simulink library "ASEToolBox2023a"  (R2023a)
settings: Solver=ode45  StartTime=0.0  StopTime=10.0  RelTol=1e-3  EnableMultiTasking=on
values from neighbouring files (symbols this model uses):
  dt = get_param(gcbh, 'g_output_datatype')    [maskSysComCallbacks_Receive.m]    (also in maskSysComCallbacks_Send.m = get_param(gcbh, 'g_input_datatype'))
undefined symbols (not defined in the file or in its folder): dCx, dCy, dCz, DiscIntNeverNeededParam, Discrete, dmassX, dmassY, dmassZ, dMx, dMy, dMz, dp, dp0, dp1, dp2, dp3, lmd_high, lmd_low, magnitude, Newton, p0, p1, p2, p3, p4, phi0, phi000, phi1, phi2, phi3, phi4, r1, r2, r3, r4, Raphson, theta0, theta1, theta2, theta3, theta4, Time, u0, u1, u2, u3, v0, v0_max, v0_min, v1, v111, v2, v222, v3, v333, v4, W1, w1, w2, W2 ... (+2)
libraries: simulink x38, etargetslib x28, simulink_extras x5, slpidlib x2, ctrlSharedLib x2, aerolibatmos2 x1, aerolibconvert2 x1, aerolibtransform2 x1, sharedtransform x1, dspstat3 x1, dspsolvers x1
(part 2 of 6)

== system ASEToolBox2023a/Aerocraft Model/ACE Guidance and Control Algorithm ==
  Time : Inport
  Eular : Inport  Port=2
  Wxyz1 : Inport  Port=3
  H : Inport  Port=4
  Add : Sum  Inputs=+-
  Add1 : Sum  Inputs=+-
  Add2 : Sum  Inputs=+-
  Add3 : Sum
  DeltaXC : Constant  Value=0
  DeltaYC : Constant  Value=0
  Discrete Transfer Fcn : DiscreteTransferFcn  Numerator=[0.0309]  Denominator=[1 -0.9691]
  Gain : Gain  Gain=0
  Gain1 : Gain
  Gain2 : Gain
  Lookup Table : Lookup  InitFcn=|  InputValues=phi000(:,1)  Table=phi000(:,2)  SaturateOnIntegerOverflow=off
      | phi00=[0.0 	60
      | 0.5 	53.175
      | 1.0 	47.6
      | 1.5 	43.275
      | 2.0 	40.2
      | 2.5 	39.1055
      | 3.0 	38.012
      | 3.5 	36.9195
      | 4.0 	35.828
      | 4.5 	34.7375
      | 5.0 	33.648
      | 5.5 	32.5595
      | 6.0 	31.472
      | 6.5 	30.3855
      | 7.0 	29.3
      | 7.5 	28.2155
      | 8.0 	27.132
      | 8.5 	26.0495
      | 9.0 	24.968
      | 9.5 	23.8875
      | 10.0 	22.808
      | 10.5 	21.7295
      | 11.0 	20.652
      | 11.5 	19.5755
      | 12.0 	18.5
      | 12.5 	17.4255
      | 13.0 	16.352
      | 13.5 	15.2795
      | 14.0 	14.208
      | 14.5 	13.1375
      | 15.0 	12.068
      | 15.5 	10.9995
      | 16.0 	9.932
      | 16.5 	8.8655
      | 17.0 	7.8
      | 17.5 	6.7355
      | 18.0 	5.672
      | 18.5 	4.6095
      | 19.0 	3.548
      | 19.5 	2.4875
      | 20.0 	1.428
      | 20.5 	0.3695
      | 21.0 	-0.688
      | 21.5 	-1.7445
      | 22.0 	-2.8
      | 22.5 	-3.8545
      | 23.0 	-4.908
      | 23.5 	-5.9605
      | 24.0 	-7.012
      | 24.5 	-8.0625
      | 25.0 	-9.112
      | 25.5 	-10.1605
      | 26.0 	-11.208
      | 26.5 	-12.2545
      | 27.0 	-13.3
      | 27.5 	-14.3445
      | 28.0 	-15.388
      | 28.5 	-14.862975
      | 29.0 	-14.3379
      | 29.5 	-13.812775
      | 30.0 	-13.2876
      | 30.5 	-12.762375
      | 31.0 	-12.2371
      | 31.5 	-11.711775
      | 32.0 	-11.1864
      | 32.5 	-10.660975
      | 33.0 	-10.1355
      | 33.5 	-9.609975
      | 34.0 	-9.0844
      | 34.5 	-8.558775
      | 35.0 	-8.0331
      | 35.5 	-7.507375
      | 36.0 	-6.9816
      | 36.5 	-6.455775
      | 37.0 	-5.9299
      | 37.5 	-5.403975
      | 38.0 	-4.878
      | 38.5 	-4.351975
      | 39.0 	-3.8259
      | 39.5 	-3.299775
      | 40.0 	-2.7736
      | 40.5 	-2.247375
      | 41.0 	-1.7211
      | 41.5 	-1.194775
      | 42.0 	-0.6684
      | 42.5 	-0.141975
      | 43.0 	0.3845
      | 43.5 	0.911025
      | 44.0 	1.4376
      | 44.5 	1.964225
      | 45.0 	2.4909
      | 45.5 	3.0167
      | 46.0 	3.01485
      | 46.5 	3.0133
      | 47.0 	3.01205
      | 47.5 	3.0111
      | 48.0 	3.01045
      | 48.5 	3.0101
      | 49.0 	3.01005
      | 49.5 	3.0103
      | 50.0 	3.01085
      | 50.5 	3.0117
      | 51.0 	3.01285
      | 51.5 	3.0143
      | 52.0 	3.01605
      | 52.5 	3.0181
      | 53.0 	3.02045
      | 53.5 	3.0231
      | 54.0 	3.02605
      | 54.5 	3.0293
      | 55.0 	3.03285
      | 55.5 	3.0367
      | 56.0 	3.04085
      | 56.5 	3.0453
      | 57.0 	3.05005
      | 57.5 	3.0551
      | 58.0 	3.06045
      | 58.5 	3.0661
      | 59.0 	3.07205
      | 59.5 	3.0783
      | 60.0 	3.08485
      | 60.5 	3.0917
      | 61.0 	3.09885
      | 61.5 	3.1063
      | 62.0 	3.11405
      | 62.5 	3.1221
      | 63.0 	3.13045
      | 63.5 	3.1391
      | 64.0 	3.14805
      | 64.5 	3.1573
      | 65.0 	3.16685
      | 65.5 	3.1767
      | 66.0 	3.18685
      | 66.5 	3.1973
      | 67.0 	3.20805
      | 67.5 	3.2191
      | 68.0 	3.23045
      | 68.5 	3.2421
      | 69.0 	3.25405
      | 69.5 	3.2663
      | 70.0 	3.27885
      | 70.5 	3.2917
      | 71.0 	3.30485
      | 71.5 	3.3183
      | 72.0 	3.33205
      | 72.5 	3.3461
      | 73.0 	3.36045
      | 73.5 	3.3751
      | 74.0 	3.39005
      | 74.5 	3.4053
      | 75.0 	3.42085
      | 75.5 	3.4367
      | 76.0 	3.45285
      | 76.5 	3.4693
      | 77.0 	3.48605
      | 77.5 	3.5031
      | 78.0 	3.52045
      | 78.5 	3.5381
      | 79.0 	3.55605
      | 79.5 	3.5743
      | 80.0 	3.59285
      | 80.5 	3.6117
      | 81.0 	3.63085
      | 81.5 	3.6503
      | 82.0 	3.67005
      | 82.5 	3.6901
      | 83.0 	3.71045
      | 83.5 	3.7311
      | 84.0 	3.75205
      | 84.5 	3.7733
      | 85.0 	3.79485
      | 85.5 	3.8167
      | 86.0 	3.83885
      | 86.5 	3.8613
      | 87.0 	3.88405
      | 87.5 	3.9071
      | 88.0 	3.93045
      | 88.5 	3.9541
      | 89.0 	3.97805
      | 89.5 	4.0023
      | 90.0 	4.02685
      | 90.5 	4.0517
      | 91.0 	4.07685
      | 91.5 	4.1023
      | 92.0 	4.12805
      | 92.5 	4.1541
      | 93.0 	4.18045
      | 93.5 	4.2071
      | 94.0 	4.23405
      | 94.5 	4.2613
      | 95.0 	4.28885
      | 95.5 	4.3167
      | 96.0 	4.34485
      | 96.5 	4.3733
      | 97.0 	4.40205
      | 97.5 	4.4311
      | 98.0 	4.46045
      | 98.5 	4.4901
      | 99.0 	4.52005
      | 99.5 	4.5503
      | 100.0 	4.5808
      | 100.5 	5.4608
      | 101.0 	6.3008
      | 101.5 	7.1008
      | 102.0 	7.8608
      | 102.5 	8.5808
      | 103.0 	9.2608
      | 103.5 	9.9008
      | 104.0 	10.5008
      | 104.5 	11.0608
      | 105.0 	11.5808
      | 105.5 	12.0608
      | 106.0 	12.5008
      | 106.5 	12.9008
      | 107.0 	13.2608
      | 107.5 	13.5808
      | 108.0 	13.8608
      | 108.5 	14.1008
      | 109.0 	14.3008
      | 109.5 	14.4608
      | 110.0 	14.5808
      | 110.5 	14.6608
      | 111.0 	14.7008
      | 111.5 	14.7008
      | 112.0 	14.6608
      | 112.5 	14.5808
      | 113.0 	14.4608
      | 113.5 	14.3008
      | 114.0 	14.1008
      | 114.5 	13.8608
      | 115.0 	13.5808
      | 115.5 	13.2608
      | 116.0 	12.9008
      | 116.5 	12.5008
      | 117.0 	12.0608
      | 117.5 	11.5808
      | 118.0 	11.0608
      | 118.5 	10.5008
      | 119.0 	9.9008
      | 119.5 	9.2608
      | 120.0 	8.5808
      | 120.5 	7.8608
      | 121.0 	7.1008
      | 121.5 	6.3008
      | 122.0 	5.4608
      | 122.5 	4.5808
      | 123.0 	3.6608
      | 123.5 	2.7008
      | 124.0 	1.7008
      | 124.5 	0.6608
      | 125.0 	-0.4192
      | 125.5 	-1.5392
      | 126.0 	-2.6992
      | 126.5 	-3.8992
      | 127.0 	-5.1392
      | 127.5 	-6.4192
      | 128.0 	-7.7392
      | 128.5 	-9.0992
      | 129.0 	-10.4992
      | 129.5 	-11.9392
      | 130.0 	-13.4192
      | 130.5 	-14.9392
      | 131.0 	-16.4992
      | 131.5 	-18.0992
      | 132.0 	-19.7392
      | 132.5 	-21.4192
      | 133.0 	-23.1392
      | 133.5 	-24.8992
      | 134.0 	-26.6992
      | 134.5 	-28.5392
      | 135.0 	-30.4192
      | 135.5 	-32.3392
      | 136.0 	-34.2992
      | 136.5 	-36.2992
      | 137.0 	-38.3392
      | 137.5 	-40.4192];
  Lookup Table1 : Lookup  InitFcn=|  InputValues=[0:1:137]  Table=|  SaturateOnIntegerOverflow=off
      InitFcn=|
      | phi00=[0.0 	60
      | 0.5 	53.175
      | 1.0 	47.6
      | 1.5 	43.275
      | 2.0 	40.2
      | 2.5 	39.1055
      | 3.0 	38.012
      | 3.5 	36.9195
      | 4.0 	35.828
      | 4.5 	34.7375
      | 5.0 	33.648
      | 5.5 	32.5595
      | 6.0 	31.472
      | 6.5 	30.3855
      | 7.0 	29.3
      | 7.5 	28.2155
      | 8.0 	27.132
      | 8.5 	26.0495
      | 9.0 	24.968
      | 9.5 	23.8875
      | 10.0 	22.808
      | 10.5 	21.7295
      | 11.0 	20.652
      | 11.5 	19.5755
      | 12.0 	18.5
      | 12.5 	17.4255
      | 13.0 	16.352
      | 13.5 	15.2795
      | 14.0 	14.208
      | 14.5 	13.1375
      | 15.0 	12.068
      | 15.5 	10.9995
      | 16.0 	9.932
      | 16.5 	8.8655
      | 17.0 	7.8
      | 17.5 	6.7355
      | 18.0 	5.672
      | 18.5 	4.6095
      | 19.0 	3.548
      | 19.5 	2.4875
      | 20.0 	1.428
      | 20.5 	0.3695
      | 21.0 	-0.688
      | 21.5 	-1.7445
      | 22.0 	-2.8
      | 22.5 	-3.8545
      | 23.0 	-4.908
      | 23.5 	-5.9605
      | 24.0 	-7.012
      | 24.5 	-8.0625
      | 25.0 	-9.112
      | 25.5 	-10.1605
      | 26.0 	-11.208
      | 26.5 	-12.2545
      | 27.0 	-13.3
      | 27.5 	-14.3445
      | 28.0 	-15.388
      | 28.5 	-14.862975
      | 29.0 	-14.3379
      | 29.5 	-13.812775
      | 30.0 	-13.2876
      | 30.5 	-12.762375
      | 31.0 	-12.2371
      | 31.5 	-11.711775
      | 32.0 	-11.1864
      | 32.5 	-10.660975
      | 33.0 	-10.1355
      | 33.5 	-9.609975
      | 34.0 	-9.0844
      | 34.5 	-8.558775
      | 35.0 	-8.0331
      | 35.5 	-7.507375
      | 36.0 	-6.9816
      | 36.5 	-6.455775
      | 37.0 	-5.9299
      | 37.5 	-5.403975
      | 38.0 	-4.878
      | 38.5 	-4.351975
      | 39.0 	-3.8259
      | 39.5 	-3.299775
      | 40.0 	-2.7736
      | 40.5 	-2.247375
      | 41.0 	-1.7211
      | 41.5 	-1.194775
      | 42.0 	-0.6684
      | 42.5 	-0.141975
      | 43.0 	0.3845
      | 43.5 	0.911025
      | 44.0 	1.4376
      | 44.5 	1.964225
      | 45.0 	2.4909
      | 45.5 	3.0167
      | 46.0 	3.01485
      | 46.5 	3.0133
      | 47.0 	3.01205
      | 47.5 	3.0111
      | 48.0 	3.01045
      | 48.5 	3.0101
      | 49.0 	3.01005
      | 49.5 	3.0103
      | 50.0 	3.01085
      | 50.5 	3.0117
      | 51.0 	3.01285
      | 51.5 	3.0143
      | 52.0 	3.01605
      | 52.5 	3.0181
      | 53.0 	3.02045
      | 53.5 	3.0231
      | 54.0 	3.02605
      | 54.5 	3.0293
      | 55.0 	3.03285
      | 55.5 	3.0367
      | 56.0 	3.04085
      | 56.5 	3.0453
      | 57.0 	3.05005
      | 57.5 	3.0551
      | 58.0 	3.06045
      | 58.5 	3.0661
      | 59.0 	3.07205
      | 59.5 	3.0783
      | 60.0 	3.08485
      | 60.5 	3.0917
      | 61.0 	3.09885
      | 61.5 	3.1063
      | 62.0 	3.11405
      | 62.5 	3.1221
      | 63.0 	3.13045
      | 63.5 	3.1391
      | 64.0 	3.14805
      | 64.5 	3.1573
      | 65.0 	3.16685
      | 65.5 	3.1767
      | 66.0 	3.18685
      | 66.5 	3.1973
      | 67.0 	3.20805
      | 67.5 	3.2191
      | 68.0 	3.23045
      | 68.5 	3.2421
      | 69.0 	3.25405
      | 69.5 	3.2663
      | 70.0 	3.27885
      | 70.5 	3.2917
      | 71.0 	3.30485
      | 71.5 	3.3183
      | 72.0 	3.33205
      | 72.5 	3.3461
      | 73.0 	3.36045
      | 73.5 	3.3751
      | 74.0 	3.39005
      | 74.5 	3.4053
      | 75.0 	3.42085
      | 75.5 	3.4367
      | 76.0 	3.45285
      | 76.5 	3.4693
      | 77.0 	3.48605
      | 77.5 	3.5031
      | 78.0 	3.52045
      | 78.5 	3.5381
      | 79.0 	3.55605
      | 79.5 	3.5743
      | 80.0 	3.59285
      | 80.5 	3.6117
      | 81.0 	3.63085
      | 81.5 	3.6503
      | 82.0 	3.67005
      | 82.5 	3.6901
      | 83.0 	3.71045
      | 83.5 	3.7311
      | 84.0 	3.75205
      | 84.5 	3.7733
      | 85.0 	3.79485
      | 85.5 	3.8167
      | 86.0 	3.83885
      | 86.5 	3.8613
      | 87.0 	3.88405
      | 87.5 	3.9071
      | 88.0 	3.93045
      | 88.5 	3.9541
      | 89.0 	3.97805
      | 89.5 	4.0023
      | 90.0 	4.02685
      | 90.5 	4.0517
      | 91.0 	4.07685
      | 91.5 	4.1023
      | 92.0 	4.12805
      | 92.5 	4.1541
      | 93.0 	4.18045
      | 93.5 	4.2071
      | 94.0 	4.23405
      | 94.5 	4.2613
      | 95.0 	4.28885
      | 95.5 	4.3167
      | 96.0 	4.34485
      | 96.5 	4.3733
      | 97.0 	4.40205
      | 97.5 	4.4311
      | 98.0 	4.46045
      | 98.5 	4.4901
      | 99.0 	4.52005
      | 99.5 	4.5503
      | 100.0 	4.5808
      | 100.5 	5.4608
      | 101.0 	6.3008
      | 101.5 	7.1008
      | 102.0 	7.8608
      | 102.5 	8.5808
      | 103.0 	9.2608
      | 103.5 	9.9008
      | 104.0 	10.5008
      | 104.5 	11.0608
      | 105.0 	11.5808
      | 105.5 	12.0608
      | 106.0 	12.5008
      | 106.5 	12.9008
      | 107.0 	13.2608
      | 107.5 	13.5808
      | 108.0 	13.8608
      | 108.5 	14.1008
      | 109.0 	14.3008
      | 109.5 	14.4608
      | 110.0 	14.5808
      | 110.5 	14.6608
      | 111.0 	14.7008
      | 111.5 	14.7008
      | 112.0 	14.6608
      | 112.5 	14.5808
      | 113.0 	14.4608
      | 113.5 	14.3008
      | 114.0 	14.1008
      | 114.5 	13.8608
      | 115.0 	13.5808
      | 115.5 	13.2608
      | 116.0 	12.9008
      | 116.5 	12.5008
      | 117.0 	12.0608
      | 117.5 	11.5808
      | 118.0 	11.0608
      | 118.5 	10.5008
      | 119.0 	9.9008
      | 119.5 	9.2608
      | 120.0 	8.5808
      | 120.5 	7.8608
      | 121.0 	7.1008
      | 121.5 	6.3008
      | 122.0 	5.4608
      | 122.5 	4.5808
      | 123.0 	3.6608
      | 123.5 	2.7008
      | 124.0 	1.7008
      | 124.5 	0.6608
      | 125.0 	-0.4192
      | 125.5 	-1.5392
      | 126.0 	-2.6992
      | 126.5 	-3.8992
      | 127.0 	-5.1392
      | 127.5 	-6.4192
      | 128.0 	-7.7392
      | 128.5 	-9.0992
      | 129.0 	-10.4992
      | 129.5 	-11.9392
      | 130.0 	-13.4192
      | 130.5 	-14.9392
      | 131.0 	-16.4992
      | 131.5 	-18.0992
      | 132.0 	-19.7392
      | 132.5 	-21.4192
      | 133.0 	-23.1392
      | 133.5 	-24.8992
      | 134.0 	-26.6992
      | 134.5 	-28.5392
      | 135.0 	-30.4192
      | 135.5 	-32.3392
      | 136.0 	-34.2992
      | 136.5 	-36.2992
      | 137.0 	-38.3392
      | 137.5 	-40.4192];
      Table=|
      | [0.00100000000000000
      | 22.7202248122665
      | 58.3064038619666
      | 104.765492770007
      | 162.824418814433
      | 232.667819078269
      | 313.266103630312
      | 395.468021527430
      | 471.038546102105
      | 540.030378965918
      | 602.628722008517
      | 659.023857898139
      | 709.384407815495
      | 753.850828206288
      | 792.533252070725
      | 825.510430148541
      | 852.448153278113
      | 873.112540037760
      | 887.733723507122
      | 896.530500155997
      | 899.691438356797
      | 897.371185606301
      | 889.689990599990
      | 876.734125941490
      | 858.556690371314
      | 835.178673785175
      | 806.590260807927
      | 772.752368466265
      | 733.598415651863
      | 690.355754501655
      | 647.183548644875
      | 605.836807012603
      | 566.814698954349
      | 530.303708451959
      | 496.408187115900
      | 465.204340032767
      | 436.752720416363
      | 411.101460882596
      | 388.286404629371
      | 368.331551311942
      | 351.249575033728
      | 337.042143519784
      | 325.700203143571
      | 317.204266573569
      | 311.525025914053
      | 308.623791335923
      | 308.375972391762
      | 309.467237850523
      | 310.761205367399
      | 311.996816815369
      | 313.121905913981
      | 314.129063812481
      | 315.020535699730
      | 315.800610414183
      | 316.473949468186
      | 317.045217261705
      | 317.519000212617
      | 317.899790794398
      | 318.191986237200
      | 318.399890510871
      | 318.528080075057
      | 318.581868019889
      | 318.566120718611
      | 318.485122236373
      | 318.342903417862
      | 318.143371350566
      | 317.890343103383
      | 317.587555621433
      | 317.238669550788
      | 316.847271438545
      | 316.416875435176
      | 315.950924791109
      | 315.452793227059
      | 314.925786202907
      | 314.373142095505
      | 313.798033291848
      | 313.203567202783
      | 312.592787201928
      | 311.968673494142
      | 311.334143917659
      | 310.692054683750
      | 310.045201057571
      | 309.396317983661
      | 308.748129198105
      | 308.103847941556
      | 307.466610971644
      | 306.839192745089
      | 306.224212640669
      | 305.624201990765
      | 305.041624229996
      | 304.478881169664
      | 303.938315122698
      | 303.422209764180
      | 302.932790589879
      | 302.472225233154
      | 302.042623720179
      | 301.646038688940
      | 301.284465580936
      | 300.959842809355
      | 300.674051905913
      | 300.428917647960
      | 300.698018161049
      | 303.000152667117
      | 307.850355275680
      | 315.143524756215
      | 324.572447991837
      | 335.769079457351
      | 348.354385617033
      | 361.957474729997
      | 376.223880747294
      | 390.819613207444
      | 405.433216636211
      | 419.776782652067
      | 433.586381240142
      | 446.620708796908
      | 458.659629694913
      | 469.502313128659
      | 478.964787061229
      | 486.876962843877
      | 493.079157212923
      | 497.418128923166
      | 499.742647647332
      | 499.898620622673
      | 497.723817719732
      | 493.042767576605
      | 485.661545355872
      | 475.360212858649
      | 461.886636970637
      | 444.952258275500
      | 424.226013339850
      | 399.327076155542
      | 369.823258573094
      | 335.223671378567
      | 294.978344407993
      | 248.477342859821
      | 195.056308059546
      | 133.999530370317
      | 64.5528584234877]
  Mux3 : Mux  Inputs=3
  PID Controller1 : slpidlib/PID Controller  Controller=PID  Form=Parallel  TimeDomain=Discrete-time  UseExternalTs=off  SampleTime=0.0100000000000000002  IntegratorMethod=Forward Euler  FilterMethod=Forward Euler  ControllerParametersSource=internal  P=1  I=0.001  UseKiTs=off  D=0  N=63.212055882855765  UseFilter=on  TunerSelectOption=Transfer Function Based (PID Tuner App)  InitialConditionSource=internal  InitialConditionForIntegrator=0  InitialConditionForFilter=0  DifferentiatorICPrevScaledInput=0  ExternalReset=none  TrackingMode=off  Kt=1  LimitOutput=off  SatLimitsSource=internal  UpperSaturationLimit=inf  LowerSaturationLimit=-inf  LinearizeAsGain=off  AntiWindupMode=none  Kb=1  LimitIntegrator=off  UpperIntegratorSaturationLimit=inf  LowerIntegratorSaturationLimit=-inf  POutMin=[]  POutMax=[]  IOutMin=[]  IOutMax=[]  DOutMin=[]  DOutMax=[]  NOutMin=[]  NOutMax=[]  SumOutMin=[]  SumOutMax=[]  SaturationOutMin=[]  SaturationOutMax=[]  PParamMin=[]  PParamMax=[]  IParamMin=[]  IParamMax=[]  DParamMin=[]  DParamMax=[]  NParamMin=[]  NParamMax=[]  KbParamMin=[]  KbParamMax=[]  KtParamMin=[]  KtParamMax=[]  KbOutMin=[]  KbOutMax=[]  KtOutMin=[]  KtOutMax=[]  IntegratorOutMin=[]  IntegratorOutMax=[]  FilterOutMin=[]  FilterOutMax=[]  SumI1OutMin=[]  SumI1OutMax=[]  SumI2OutMin=[]  SumI2OutMax=[]  SumI3OutMin=[]  SumI3OutMax=[]  SumI4OutMin=[]  SumI4OutMax=[]  SumDOutMin=[]  SumDOutMax=[]  DifferentiatorOutMin=[]  DifferentiatorOutMax=[]  FilterDiffOutCoefMin=[]  FilterDiffOutCoefMax=[]  ReciprocalOutMin=[]  ReciprocalOutMax=[]  SumDenOutMin=[]  SumDenOutMax=[]  SumNumOutMin=[]  SumNumOutMax=[]  DivideOutMin=[]  DivideOutMax=[]  UdiffTsProdOutMin=[]  UdiffTsProdOutMax=[]  NTsProdOutMin=[]  NTsProdOutMax=[]  UintegralTsProdOutMin=[]  UintegralTsProdOutMax=[]  UngainTsProdOutMin=[]  UngainTsProdOutMax=[]  ClampingZeroOutDataTypeStr=Inherit: Inherit via back propagation  ClampingZeroOutMin=[]  ClampingZeroOutMax=[]  FilterDenConstantOutDataTypeStr=Inherit: Inherit via back propagation  FilterDenConstantOutMin=[]  FilterDenConstantOutMax=[]  PCopyOutDataTypeStr=Inherit: Inherit via back propagation  PCopyOutMin=[]  PCopyOutMax=[]  NCopyOutDataTypeStr=Inherit: Inherit via back propagation  NCopyOutMin=[]  NCopyOutMax=[]  IntegratorContinuousStateAttributes=''  IntegratorStateMustResolveToSignalObject=off  IntegratorRTWStateStorageClass=Auto  FilterContinuousStateAttributes=''  FilterStateMustResolveToSignalObject=off  FilterRTWStateStorageClass=Auto  ParallelPVariant=InternalParameters  IdealPVariant=Disabled  IVariant=InternalParameters  DVariant=InternalParameters  IntegratorVariant=Discrete  SatVariant=Disabled  AWVariant=Passthrough  PCopyVariant=Disabled  TRVariant=Disabled  FdbkBlocksVariant=Forward  IdealPFdbkVariant=Disabled  SatFdbkVariant=Disabled  DerivativeFilterVariant=ForwardEulerFilter  NVariant=InternalParameters  NCopyVariant=Disabled  FilterICVariant=InternalICsFilter  IntegratorICVariant=InternalICs  ExternalResetVariant=Disabled  TRSumVariant=Passthrough  SumFdbkVariant=Disabled  SumVariant=Sum_PID  TsampFilterVariant=InternalTs  TsampNgainVariant=Passthrough  TsampIntegralVariant=Disabled_SignalSpec  ExternalSaturationOutDataTypeStr=Inherit: Same as second input
  PID Controller2 : slpidlib/PID Controller  Controller=PID  Form=Parallel  TimeDomain=Discrete-time  UseExternalTs=off  SampleTime=0.0100000000000000002  IntegratorMethod=Forward Euler  FilterMethod=Forward Euler  ControllerParametersSource=internal  P=0.02  I=0.080000000000000  UseKiTs=off  D=0.006  N=63.212055882855765  UseFilter=on  TunerSelectOption=Transfer Function Based (PID Tuner App)  InitialConditionSource=internal  InitialConditionForIntegrator=0  InitialConditionForFilter=0  DifferentiatorICPrevScaledInput=0  ExternalReset=none  TrackingMode=off  Kt=1  LimitOutput=off  SatLimitsSource=internal  UpperSaturationLimit=inf  LowerSaturationLimit=-inf  LinearizeAsGain=off  AntiWindupMode=none  Kb=1  LimitIntegrator=off  UpperIntegratorSaturationLimit=inf  LowerIntegratorSaturationLimit=-inf  POutMin=[]  POutMax=[]  IOutMin=[]  IOutMax=[]  DOutMin=[]  DOutMax=[]  NOutMin=[]  NOutMax=[]  SumOutMin=[]  SumOutMax=[]  SaturationOutMin=[]  SaturationOutMax=[]  PParamMin=[]  PParamMax=[]  IParamMin=[]  IParamMax=[]  DParamMin=[]  DParamMax=[]  NParamMin=[]  NParamMax=[]  KbParamMin=[]  KbParamMax=[]  KtParamMin=[]  KtParamMax=[]  KbOutMin=[]  KbOutMax=[]  KtOutMin=[]  KtOutMax=[]  IntegratorOutMin=[]  IntegratorOutMax=[]  FilterOutMin=[]  FilterOutMax=[]  SumI1OutMin=[]  SumI1OutMax=[]  SumI2OutMin=[]  SumI2OutMax=[]  SumI3OutMin=[]  SumI3OutMax=[]  SumI4OutMin=[]  SumI4OutMax=[]  SumDOutMin=[]  SumDOutMax=[]  DifferentiatorOutMin=[]  DifferentiatorOutMax=[]  FilterDiffOutCoefMin=[]  FilterDiffOutCoefMax=[]  ReciprocalOutMin=[]  ReciprocalOutMax=[]  SumDenOutMin=[]  SumDenOutMax=[]  SumNumOutMin=[]  SumNumOutMax=[]  DivideOutMin=[]  DivideOutMax=[]  UdiffTsProdOutMin=[]  UdiffTsProdOutMax=[]  NTsProdOutMin=[]  NTsProdOutMax=[]  UintegralTsProdOutMin=[]  UintegralTsProdOutMax=[]  UngainTsProdOutMin=[]  UngainTsProdOutMax=[]  ClampingZeroOutDataTypeStr=Inherit: Inherit via back propagation  ClampingZeroOutMin=[]  ClampingZeroOutMax=[]  FilterDenConstantOutDataTypeStr=Inherit: Inherit via back propagation  FilterDenConstantOutMin=[]  FilterDenConstantOutMax=[]  PCopyOutDataTypeStr=Inherit: Inherit via back propagation  PCopyOutMin=[]  PCopyOutMax=[]  NCopyOutDataTypeStr=Inherit: Inherit via back propagation  NCopyOutMin=[]  NCopyOutMax=[]  IntegratorContinuousStateAttributes=''  IntegratorStateMustResolveToSignalObject=off  IntegratorRTWStateStorageClass=Auto  FilterContinuousStateAttributes=''  FilterStateMustResolveToSignalObject=off  FilterRTWStateStorageClass=Auto  ParallelPVariant=InternalParameters  IdealPVariant=Disabled  IVariant=InternalParameters  DVariant=InternalParameters  IntegratorVariant=Discrete  SatVariant=Disabled  AWVariant=Passthrough  PCopyVariant=Disabled  TRVariant=Disabled  FdbkBlocksVariant=Forward  IdealPFdbkVariant=Disabled  SatFdbkVariant=Disabled  DerivativeFilterVariant=ForwardEulerFilter  NVariant=InternalParameters  NCopyVariant=Disabled  FilterICVariant=InternalICsFilter  IntegratorICVariant=InternalICs  ExternalResetVariant=Disabled  TRSumVariant=Passthrough  SumFdbkVariant=Disabled  SumVariant=Sum_PID  TsampFilterVariant=InternalTs  TsampNgainVariant=Passthrough  TsampIntegralVariant=Disabled_SignalSpec  ExternalSaturationOutDataTypeStr=Inherit: Same as second input
  Rate Limiter : RateLimiter  RisingSlewLimit=100  FallingSlewLimit=-100  SampleTimeMode=inherited
  Saturation : Saturate  UpperLimit=15  LowerLimit=-15
  Scope{,1..3} (4 alike) : Scope
  Selector : Selector  InputPortWidth=3  IndexOptions=Index vector (dialog)  Indices=1  OutputSizes=1
  Selector1 : Selector  InputPortWidth=3  IndexOptions=Index vector (dialog)  Indices=3  OutputSizes=1
  DeltaXYZC : Outport
  wires:
  Add3/1 -> Add/1
  Add/1 -> Scope2/1, PID Controller1/1
  Add2/1 -> Gain/1
  Gain/1 -> Add3/1
  Lookup Table1/1 -> Add2/1
  H/1 -> Add2/2
  PID Controller1/1 -> Gain2/1
  Selector1/1 -> Add1/2  "Wz"
  Add1/1 -> Scope1/1, PID Controller2/1
  Wxyz1/1 -> Selector1/1
  Mux3/1 -> Discrete Transfer Fcn/1
  Time/1 -> Lookup Table/1, Lookup Table1/1
  Lookup Table/1 -> Scope/1, Add3/2  "phi*"
  Eular/1 -> Selector/1
  DeltaYC/1 -> Mux3/2  "DeltaYC"
  DeltaXC/1 -> Mux3/1  "DeltaXC"
  Selector/1 -> Scope3/1, Add/2  "phi"
  PID Controller2/1 -> Gain1/1
  Saturation/1 -> Rate Limiter/1
  Rate Limiter/1 -> Mux3/3  "DeltaZC"
  Gain1/1 -> Saturation/1
  Gain2/1 -> Add1/1
  Discrete Transfer Fcn/1 -> DeltaXYZC/1

== system ASEToolBox2023a/Aerocraft Model/ACE Mass ==
  Time : Inport
  Add : Sum  Inputs=|+++|
  Add1 : Sum  Inputs=+-
  Add2 : Sum  Inputs=+-
  Constant0 : Constant  Value=0
  Constant00 : Constant  Value=0
  Divide1 : Product  Inputs=/*
  Divide2 : Product  Inputs=/*
  Gain1 : Gain  Gain=-1
  Gain2 : Gain  Gain=-1
  Integrator1 : Integrator  InitialConditionSource=external
  Integrator2 : Integrator  InitialConditionSource=external
  Switch1 : Switch  SaturateOnIntegerOverflow=off  InputSameDT=off
  Switch2 : Switch  SaturateOnIntegerOverflow=off  InputSameDT=off
  Time1 : Constant  Value=6
  Time2 : Constant  Value=15
  m0 : Constant  Value=110
  m1 : Constant  Value=8
  m2 : Constant  Value=4
  m : Outport
  wires:
  Constant00/1 -> Switch2/1
  Integrator2/1 -> Switch2/3
  Constant0/1 -> Switch1/1
  Integrator1/1 -> Switch1/3
  m1/1 -> Integrator1/2, Divide1/2
  m2/1 -> Integrator2/2, Divide2/2
  Add/1 -> m/1
  Time1/1 -> Divide1/1, Add1/2
  Divide1/1 -> Gain1/1
  Gain1/1 -> Integrator1/1
  Time2/1 -> Divide2/1, Add2/2
  Divide2/1 -> Gain2/1
  Gain2/1 -> Integrator2/1
  Time/1 -> Add1/1, Add2/1
  Switch1/1 -> Add/1
  Add1/1 -> Switch1/2
  Switch2/1 -> Add/3
  Add2/1 -> Switch2/2
  m0/1 -> Add/2

== system ASEToolBox2023a/Aerocraft Model/ACE Propulsion ==
  Time : Inport
  Add : Sum
  Add1 : Sum  Inputs=+-
  Add2 : Sum  Inputs=+-
  Constant0 : Constant  Value=0
  P1 : Constant  Value=3280
  P2 : Constant  Value=420
  Switch1 : Switch  SaturateOnIntegerOverflow=off  InputSameDT=off
  Switch2 : Switch  SaturateOnIntegerOverflow=off  InputSameDT=off
  Time1 : Constant  Value=6
  Time2 : Constant  Value=15
  P : Outport
  wires:
  Switch1/1 -> P/1
  Time/1 -> Add1/1, Add2/1
  Time1/1 -> Add1/2
  Time2/1 -> Add2/2
  P2/1 -> Switch2/3, Add/1
  P1/1 -> Add/2
  Add/1 -> Switch1/3
  Add1/1 -> Switch1/2
  Constant0/1 -> Switch2/1
  Add2/1 -> Switch2/2
  Switch2/1 -> Switch1/1

== system ASEToolBox2023a/SIMSystemModule/ASEMonitorIn ==
  Compare To Constant : simulink/Logic and Bit Operations/Compare To Constant  relop===  const=g_iFrameType  OutDataTypeStr=boolean
  Enabled Subsystem : Subsystem  TreatAsAtomicUnit=on
  FrameCheck : Subsystem
  MonitorReceive : S-Function  Priority=6  FunctionName=UDPRecv_sfcn  Parameters=g_localip, g_localport, g_ip, g_port, g_buffersize, g_datatype, g_sample_time,g_reusePort  SFunctionDeploymentMode=off  EnableBusSupport=off  mask(UDP Receive){g_localip="192.168.0.7", g_localport=8080, g_ip="192.168.0.3", g_port=9090, g_buffersize=16, g_datatype=uint8, g_sample_time=g_sample_time, g_reusePort=1}
      mask prompts: g_localip "本机IP地址:"; g_localport "端口号:"; g_ip "远程IP地址:"; g_port "远程端口号:"; g_buffersize "接收缓存大小:"; g_datatype "数据类型:"; g_sample_time "采样时间:"; g_reusePort "收发是否都用同一个端口:"
      mask help:
      | Receive UDP packets on the host computer at the specified local port.
      |
      | The block outputs the received UDP data as a one-dimensional array of the specified data type.
      |
      | Set the Local IP port parameter to the desired port where the sender sends the UDP data. Set the Data type parameter to match the data type of the incoming UDP data. Set the Blocking time parameter to specify the duration to wait for a UDP packet before continuing.
      |
      | 注意：IP请使用双引号括起来，如"192.168.0.7"。
      mask TypeOptions g_datatype: double | single | int8 | uint8 | int16 | uint16 | int32 | uint32 | boolean
      mask DialogControl ParameterGroupVar Prompt: 参数
      mask Display:
      | port_label('output', 1, 'Data');
      | port_label('output', 2, 'Len');
  Subsystem1 : Subsystem
  Terminator{,1..2,4} (4 alike) : Terminator
  TunePara : Outport
  wires:
  Subsystem1/5(ACKFramePara) -> Enabled Subsystem/1(in)
  MonitorReceive/1 -> FrameCheck/1(In1), Subsystem1/1(In1)
  MonitorReceive/2 -> Terminator4/1
  Subsystem1/2(ACKSourceID) -> Terminator1/1
  Subsystem1/3(ACKTargetID) -> Terminator2/1
  Subsystem1/1(ACKFrameCounter) -> Terminator/1
  FrameCheck/1(Out1) -> Subsystem1/Enable
  Subsystem1/4(ACKFrameType) -> Compare To Constant/1
  Enabled Subsystem/1(out) -> TunePara/1
  Compare To Constant/1 -> Enabled Subsystem/Enable

== system ASEToolBox2023a/SIMSystemModule/ASEMonitorOut ==
  Scope : Inport
  BitCheckSum1 : Subsystem
  Byte Pack : etargetslib/Byte Pack  datatypes={'single'}  byteAlign=1
  Byte Pack1 : etargetslib/Byte Pack  datatypes={'uint16','uint16','uint32'}  byteAlign=1
  Constant : Constant  Value=g_iFrameType  OutDataTypeStr=uint8
  Constant1 : Constant  Value=hex2dec('DAA5')
  CounterFreeRunning1 : simulink/Sources/Counter Free-Running  NumBits=32  tsamp=-1
  Data Type Conversion : DataTypeConversion  OutDataTypeStr=single  SaturateOnIntegerOverflow=off  RndMeth=Floor
  Data Type Conversion1 : DataTypeConversion  OutDataTypeStr=uint8  SaturateOnIntegerOverflow=off  RndMeth=Floor
  Data Type Conversion10 : DataTypeConversion  OutDataTypeStr=uint16  SaturateOnIntegerOverflow=off  RndMeth=Floor
  Data Type Conversion11 : DataTypeConversion  OutDataTypeStr=uint32  SaturateOnIntegerOverflow=off  RndMeth=Floor
  Data Type Conversion8 : DataTypeConversion  OutDataTypeStr=uint16  SaturateOnIntegerOverflow=off  RndMeth=Floor
  MonitorSend : S-Function  Priority=0  FunctionName=UDPSend_sfcn  Parameters=g_localIP, g_localPort, g_ip, g_port, g_buffersize  SFunctionDeploymentMode=off  EnableBusSupport=off  mask(UDP Send){g_localIP="192.168.0.7", g_localPort=8080, g_ip="192.168.0.3", g_port=9090, g_buffersize=16}
      mask prompts: g_localIP "本机IP地址:"; g_localPort "本机端口:"; g_ip "远程机IP地址:"; g_port "远程机端口号:"; g_buffersize "发送缓存大小:"
      mask help: Send a UDP packet to a network address identified by the remote IP address and remote IP port parameters.
      mask DialogControl ParameterGroupVar Prompt: 参数
      mask Display: port_label('input', 1, 'Data');
  Mux3 : Mux  Inputs=5
  Mux4 : Mux  Inputs=2
  Signal Copy : SignalConversion  OverrideOpt=on
  SourceID1 : Constant  Value=hex2dec('01')  OutDataTypeStr=uint8
  TargetID1 : Constant  Value=hex2dec('12')  OutDataTypeStr=uint8
  Width1 : Width
  wires:
  Mux3/1 -> Mux4/1, BitCheckSum1/1(In1)
  Data Type Conversion8/1 -> Byte Pack1/1
  SourceID1/1 -> Mux3/2
  Width1/1 -> Data Type Conversion10/1
  Constant1/1 -> Data Type Conversion8/1
  Byte Pack/1 -> Mux3/5
  Data Type Conversion10/1 -> Byte Pack1/2
  TargetID1/1 -> Mux3/3
  Data Type Conversion11/1 -> Byte Pack1/3
  CounterFreeRunning1/1 -> Data Type Conversion11/1
  Mux4/1 -> Data Type Conversion1/1, Width1/1
  Scope/1 -> Data Type Conversion/1
  Byte Pack1/1 -> Mux3/1
  Signal Copy/1 -> MonitorSend/1  "abc"
  BitCheckSum1/1(Out1) -> Mux4/2
  Constant/1 -> Mux3/4
  Data Type Conversion/1 -> Byte Pack/1
  Data Type Conversion1/1 -> Signal Copy/1

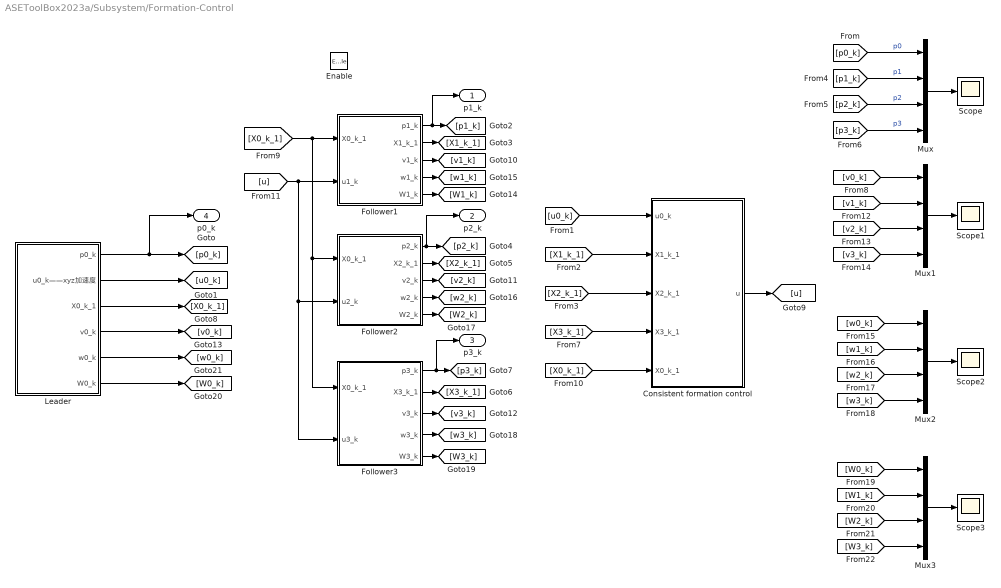
== system ASEToolBox2023a/Subsystem/Formation-Control ==
  Enable : EnablePort
  "Consistent formation control " : Subsystem
  Follower1 : Subsystem
  Follower2 : Subsystem
  Follower3 : Subsystem
  Leader : Subsystem
  Mux{,1..3} (4 alike) : Mux
  Scope{,1..3} (4 alike) : Scope
  p1_k : Outport
  p2_k : Outport  Port=2
  p3_k : Outport  Port=3
  p0_k : Outport  Port=4
  wires:
  Follower2/3(v2_k) -> [v2_k]
  Follower2/2(X2_k_1) -> [X2_k_1]
  Leader/5(w0_k) -> [w0_k]
  [X0_k_1] -> Follower3/1(X0_k_1), Follower2/1(X0_k_1), Follower1/1(X0_k_1)
  [w3_k] -> Mux2/4
  [p0_k] -> Mux/1  "p0"
  Follower3/2(X3_k_1) -> [X3_k_1]
  Mux2/1 -> Scope2/1
  Follower2/1(p2_k) -> p2_k/1, [p2_k]
  [p3_k] -> Mux/4  "p3"
  [w2_k] -> Mux2/3
  Mux1/1 -> Scope1/1
  Leader/4(v0_k) -> [v0_k]
  Follower1/1(p1_k) -> p1_k/1, [p1_k]
  [p2_k] -> Mux/3  "p2"
  Follower3/1(p3_k) -> p3_k/1, [p3_k]
  Follower1/3(v1_k) -> [v1_k]
  [p1_k] -> Mux/2  "p1"
  Follower3/4(w3_k) -> [w3_k]
  [W1_k] -> Mux3/2
  Mux/1 -> Scope/1
  [X1_k_1] -> "Consistent formation control "/2(X1_k_1)
  [v1_k] -> Mux1/2
  Follower1/2(X1_k_1) -> [X1_k_1]
  [W2_k] -> Mux3/3
  [v3_k] -> Mux1/4
  [u] -> Follower3/2(u3_k), Follower2/2(u2_k), Follower1/2(u1_k)
  [W3_k] -> Mux3/4
  [w1_k] -> Mux2/2
  [v0_k] -> Mux1/1
  [v2_k] -> Mux1/3
  [w0_k] -> Mux2/1
  Leader/2(u0_k——xyz加速度) -> [u0_k]
  Mux3/1 -> Scope3/1
  [W0_k] -> Mux3/1
  Leader/1(p0_k) -> p0_k/1, [p0_k]
  [X3_k_1] -> "Consistent formation control "/4(X3_k_1)
  [X0_k_1] -> "Consistent formation control "/5(X0_k_1)
  [X2_k_1] -> "Consistent formation control "/3(X2_k_1)
  Follower3/3(v3_k) -> [v3_k]
  Follower2/4(w2_k) -> [w2_k]
  Follower3/5(W3_k) -> [W3_k]
  [u0_k] -> "Consistent formation control "/1(u0_k)
  Follower2/5(W2_k) -> [W2_k]
  Leader/3(X0_k_1) -> [X0_k_1]
  "Consistent formation control "/1(u) -> [u]
  Follower1/5(W1_k) -> [W1_k]
  Follower1/4(w1_k) -> [w1_k]
  Leader/6(W0_k) -> [W0_k]

== system ASEToolBox2023a/Subsystem/GNC_EKF ==
  Cbn : Inport
  accl_ned_m/s2 : Inport  Port=2
  QGC_sensor_reinit : Inport  Port=3
  GPS_fixtype : Inport  Port=4
  GPS_V_m/s : Inport  Port=5
  GPS_LLA_rad : Inport  Port=6
  GPSHdop : Inport  Port=7
  Cast To Boolean : DataTypeConversion  OutDataTypeStr=double  SaturateOnIntegerOverflow=off  RndMeth=Floor
  Compare To Constant : simulink/Logic and Bit Operations/Compare To Constant  relop=>=  const=1  OutDataTypeStr=boolean
  Compare To Constant1 : simulink/Logic and Bit Operations/Compare To Constant  relop=>=  const=1  OutDataTypeStr=boolean
  GPS_Data_Process : Subsystem
  Logical Operator : Logic  AllPortsSameDT=off  OutDataTypeStr=boolean
  Translation_estimate : Subsystem
  vxy_estimout : Outport
  Pxy_estimout : Outport  Port=2
  posNE_gps : Outport  Port=3
  tag scope: AccelFusion_sta=global
  wires:
  Compare To Constant/1 -> Logical Operator/1
  GPS_Data_Process/1(init_GPSLLAflag) -> Compare To Constant1/1
  GPSHdop/1 -> Translation_estimate/6(GPSHdop), GPS_Data_Process/5(GPSHdop)
  QGC_sensor_reinit/1 -> Translation_estimate/7(QGC_init), GPS_Data_Process/4(QGC_sensor_reinit)
  GPS_LLA_rad/1 -> GPS_Data_Process/2(GPS_LLA_rad)
  GPS_V_m/s/1 -> GPS_Data_Process/1(GPS_V_m/s)
  accl_ned_m/s2/1 -> Translation_estimate/2(accl_ned_m/s2)
  Cbn/1 -> Translation_estimate/1(Cbn)
  GPS_Data_Process/2(vne_gps) -> Translation_estimate/3(vne_gps)
  GPS_Data_Process/3(posNE_gps) -> posNE_gps/1, Translation_estimate/4(posNE_gps1)
  GPS_fixtype/1 -> Compare To Constant/1, Translation_estimate/5(GPSstate), GPS_Data_Process/3(GPS_fixtype)  "sts"
  Translation_estimate/1(vxy_estimout) -> vxy_estimout/1
  Translation_estimate/2(Pxy_estimout) -> Pxy_estimout/1
  Cast To Boolean/1 -> [AccelFusion_sta]
  Compare To Constant1/1 -> Logical Operator/2
  Logical Operator/1 -> Translation_estimate/Enable, Cast To Boolean/1

== system ASEToolBox2023a/ACEModule/IMU/FrameCheck3 ==
  note: 判断前两个字节帧头、次1个字节帧长度、校验和
  In1 : Inport
  AND : Logic  Inputs=3  IconShape=distinctive  AllPortsSameDT=off  OutDataTypeStr=boolean
  Bitwise AND : simulink/Logic and Bit Operations/Bitwise Operator  logicop=AND  UseBitMask=on  BitMask=0xFF  BitMaskRealWorld=Stored Integer
      settings: LibrarySourceBlock=|
      | simulink/Quick Insert/Logic and Bit
      | Operations/Bitwise AND
  Byte Unpack1 : etargetslib/Byte Unpack  dimensions={1}  datatypes={'uint16'}  byteAlign=1
      settings: LibrarySourceBlock=embeddedtargetslib/Host Communication/Byte Unpack
  Byte Unpack3 : etargetslib/Byte Unpack  dimensions={1}  datatypes={'uint16'}  byteAlign=1
      settings: LibrarySourceBlock=embeddedtargetslib/Host Communication/Byte Unpack
  Compare To Constant : simulink/Logic and Bit Operations/Compare To Constant  relop===  const=0xDAA5  OutDataTypeStr=boolean
  Compare To Zero : simulink/Logic and Bit Operations/Compare To Zero  relop===  OutDataTypeStr=boolean
  Data Type Conversion : DataTypeConversion  OutDataTypeStr=uint32  SaturateOnIntegerOverflow=off  RndMeth=Floor
  Data Type Conversion1 : DataTypeConversion  OutDataTypeStr=uint8  SaturateOnIntegerOverflow=off  RndMeth=Floor
  Demux : Demux  Outputs=[2,2,-1]
      settings: DisplayOption=none
  Relational Operator : RelationalOperator  Operator===  OutDataTypeStr=boolean  RndMeth=Simplest  InputSameDT=off
  Sum ofElements : Sum  Inputs=+
  Terminator : Terminator
  Width : Width  DataType=uint16
  Out1 : Outport
  wires:
  AND/1 -> Out1/1
  Bitwise AND/1 -> Data Type Conversion1/1
  Demux/1 -> Byte Unpack3/1
  Compare To Constant/1 -> AND/1
  Compare To Zero/1 -> AND/3
  Width/1 -> Relational Operator/2
  Relational Operator/1 -> AND/2
  Demux/2 -> Byte Unpack1/1
  In1/1 -> Demux/1, Data Type Conversion/1, Width/1
  Data Type Conversion/1 -> Sum ofElements/1
  Byte Unpack3/1 -> Compare To Constant/1
  Demux/3 -> Terminator/1
  Data Type Conversion1/1 -> Compare To Zero/1
  Sum ofElements/1 -> Bitwise AND/1
  Byte Unpack1/1 -> Relational Operator/1

== system ASEToolBox2023a/ACEModule/IMU/Subsystem5 ==
  note: 除去帧头等12个字节之外的数据字节长度，如果为4的倍数则正常并解析为单精度，否则不进行解析（强行解析后报错）
  In1 : Inport
  Enable : EnablePort
  Byte Unpack1 : etargetslib/Byte Unpack  dimensions={1}  datatypes={'uint32'}  byteAlign=1
      settings: LibrarySourceBlock=embeddedtargetslib/Host Communication/Byte Unpack
  Byte Unpack2 : etargetslib/Byte Unpack  dimensions={1}  datatypes={'uint16'}  byteAlign=1
      settings: LibrarySourceBlock=embeddedtargetslib/Host Communication/Byte Unpack
  Compare To Zero : simulink/Logic and Bit Operations/Compare To Zero  relop===  OutDataTypeStr=boolean
  Constant : Constant  Value=4  OutDataTypeStr=uint16
  Data Type Conversion{,1..2,4} (4 alike) : DataTypeConversion  OutDataTypeStr=double  SaturateOnIntegerOverflow=off  RndMeth=Floor
  Demux : Demux  Outputs=[2,2,4,2,1,-1,1]
      settings: DisplayOption=none
  Mod : Math  Operator=mod
  Subsystem : Subsystem
  Terminator : Terminator
  Terminator1 : Terminator
  Terminator2 : Terminator
  Width : Width  DataType=uint16
  Counter : Outport
  SourceID : Outport  Port=2
  FrameType : Outport  Port=3
  Para : Outport  Port=4
  wires:
  Subsystem/1(Out1) -> Data Type Conversion/1
  Constant/1 -> Mod/2
  In1/1 -> Demux/1
  Width/1 -> Mod/1
  Demux/3 -> Byte Unpack1/1
  Data Type Conversion4/1 -> FrameType/1
  Data Type Conversion1/1 -> Counter/1
  Demux/2 -> Terminator1/1
  Demux/6 -> Subsystem/1(In1), Width/1
  Data Type Conversion2/1 -> SourceID/1
  Demux/1 -> Terminator2/1
  Data Type Conversion/1 -> Para/1
  Mod/1 -> Compare To Zero/1
  Compare To Zero/1 -> Subsystem/Enable
  Byte Unpack1/1 -> Data Type Conversion1/1
  Demux/7 -> Terminator/1
  Byte Unpack2/1 -> Data Type Conversion2/1
  Demux/5 -> Data Type Conversion4/1
  Demux/4 -> Byte Unpack2/1

== system ASEToolBox2023a/ACEModule/ServoCardPack/BitChk ==
  In1 : Inport
  Add : Sum
  Bitwise AND : simulink/Logic and Bit Operations/Bitwise Operator  logicop=AND  UseBitMask=on  BitMask=hex2dec('FF')  BitMaskRealWorld=Stored Integer
      settings: LibrarySourceBlock=|
      | simulink/Quick Insert/Logic and Bit
      | Operations/Bitwise AND
  Bitwise AND1 : simulink/Logic and Bit Operations/Bitwise Operator  logicop=AND  UseBitMask=on  BitMask=hex2dec('FF')  BitMaskRealWorld=Stored Integer
      settings: LibrarySourceBlock=|
      | simulink/Quick Insert/Logic and Bit
      | Operations/Bitwise AND
  Bitwise NOT : simulink/Logic and Bit Operations/Bitwise Operator  logicop=NOT  UseBitMask=off  BitMask=bin2dec('11011001')  BitMaskRealWorld=Stored Integer
      settings: LibrarySourceBlock=|
      | simulink/Quick Insert/Logic and Bit
      | Operations/Bitwise NOT
  Constant5 : Constant
  Data Type Conversion10 : DataTypeConversion  OutDataTypeStr=uint8  SaturateOnIntegerOverflow=off  RndMeth=Floor
  Data Type Conversion11 : DataTypeConversion  OutDataTypeStr=uint16  SaturateOnIntegerOverflow=off  RndMeth=Floor
  Data Type Conversion12 : DataTypeConversion  OutDataTypeStr=uint8  SaturateOnIntegerOverflow=off  RndMeth=Floor
  Data Type Conversion8 : DataTypeConversion  OutDataTypeStr=uint32  SaturateOnIntegerOverflow=off  RndMeth=Floor
  Data Type Conversion9 : DataTypeConversion  OutDataTypeStr=uint16  SaturateOnIntegerOverflow=off  RndMeth=Floor
  Sum of Elements : Sum  Inputs=+
  Out1 : Outport
  wires:
  Bitwise NOT/1 -> Data Type Conversion9/1
  Constant5/1 -> Data Type Conversion11/1
  Sum of Elements/1 -> Bitwise AND/1
  Bitwise AND/1 -> Data Type Conversion10/1
  Add/1 -> Bitwise AND1/1
  Data Type Conversion9/1 -> Add/1
  Data Type Conversion11/1 -> Add/2
  Data Type Conversion8/1 -> Sum of Elements/1
  Data Type Conversion10/1 -> Bitwise NOT/1
  In1/1 -> Data Type Conversion8/1
  Data Type Conversion12/1 -> Out1/1
  Bitwise AND1/1 -> Data Type Conversion12/1

== system ASEToolBox2023a/ACEModule/ServoCardUnpack/FrameCheck1 ==
  note: 判断前两个字节帧头、次1个字节帧长度、校验和
  In1 : Inport
  AND : Logic  Inputs=3  IconShape=distinctive  AllPortsSameDT=off  OutDataTypeStr=boolean
  Bitwise AND : simulink/Logic and Bit Operations/Bitwise Operator  logicop=AND  UseBitMask=on  BitMask=0xFF  BitMaskRealWorld=Stored Integer
      settings: LibrarySourceBlock=|
      | simulink/Quick Insert/Logic and Bit
      | Operations/Bitwise AND
  Byte Unpack1 : etargetslib/Byte Unpack  dimensions={1}  datatypes={'uint16'}  byteAlign=1
      settings: LibrarySourceBlock=embeddedtargetslib/Host Communication/Byte Unpack
  Byte Unpack3 : etargetslib/Byte Unpack  dimensions={1}  datatypes={'uint16'}  byteAlign=1
      settings: LibrarySourceBlock=embeddedtargetslib/Host Communication/Byte Unpack
  Compare To Constant : simulink/Logic and Bit Operations/Compare To Constant  relop===  const=0xDAA5  OutDataTypeStr=boolean
  Compare To Zero : simulink/Logic and Bit Operations/Compare To Zero  relop===  OutDataTypeStr=boolean
  Data Type Conversion : DataTypeConversion  OutDataTypeStr=uint32  SaturateOnIntegerOverflow=off  RndMeth=Floor
  Data Type Conversion1 : DataTypeConversion  OutDataTypeStr=uint8  SaturateOnIntegerOverflow=off  RndMeth=Floor
  Demux : Demux  Outputs=[2,2,-1]
      settings: DisplayOption=none
  Relational Operator : RelationalOperator  Operator===  OutDataTypeStr=boolean  RndMeth=Simplest  InputSameDT=off
  Sum ofElements : Sum  Inputs=+
  Terminator : Terminator
  Width : Width  DataType=uint16
  Out1 : Outport
  wires:
  AND/1 -> Out1/1
  Bitwise AND/1 -> Data Type Conversion1/1
  Demux/1 -> Byte Unpack3/1
  Compare To Constant/1 -> AND/1
  Width/1 -> Relational Operator/2
  Relational Operator/1 -> AND/2
  Demux/2 -> Byte Unpack1/1
  In1/1 -> Demux/1, Data Type Conversion/1, Width/1
  Data Type Conversion/1 -> Sum ofElements/1
  Byte Unpack3/1 -> Compare To Constant/1
  Demux/3 -> Terminator/1
  Sum ofElements/1 -> Bitwise AND/1
  Byte Unpack1/1 -> Relational Operator/1
  Compare To Zero/1 -> AND/3
  Data Type Conversion1/1 -> Compare To Zero/1

== system ASEToolBox2023a/ACEModule/ServoCardUnpack/Subsystem6 ==
  note: 除去帧头等12个字节之外的数据字节长度，如果为4的倍数则正常并解析为单精度，否则不进行解析（强行解析后报错）
  In1 : Inport
  Enable : EnablePort
  Byte Unpack1 : etargetslib/Byte Unpack  dimensions={1}  datatypes={'uint32'}  byteAlign=1
      settings: LibrarySourceBlock=embeddedtargetslib/Host Communication/Byte Unpack
  Byte Unpack2 : etargetslib/Byte Unpack  dimensions={1}  datatypes={'uint16'}  byteAlign=1
      settings: LibrarySourceBlock=embeddedtargetslib/Host Communication/Byte Unpack
  Compare To Zero : simulink/Logic and Bit Operations/Compare To Zero  relop===  OutDataTypeStr=boolean
  Constant : Constant  Value=4  OutDataTypeStr=uint16
  Data Type Conversion{,1..2,4} (4 alike) : DataTypeConversion  OutDataTypeStr=double  SaturateOnIntegerOverflow=off  RndMeth=Floor
  Demux : Demux  Outputs=[2,2,4,2,1,-1,1]
      settings: DisplayOption=none
  Mod : Math  Operator=mod
  Subsystem : Subsystem
  Terminator : Terminator
  Terminator1 : Terminator
  Terminator2 : Terminator
  Width : Width  DataType=uint16
  ACKFrameCounter : Outport
  ACKSourceID : Outport  Port=2
  ACKFrameType : Outport  Port=3
  ACKFramePara : Outport  Port=4
  wires:
  Subsystem/1(Out1) -> Data Type Conversion/1
  Constant/1 -> Mod/2
  In1/1 -> Demux/1
  Width/1 -> Mod/1
  Demux/3 -> Byte Unpack1/1
  Data Type Conversion4/1 -> ACKFrameType/1
  Data Type Conversion1/1 -> ACKFrameCounter/1
  Demux/2 -> Terminator1/1
  Demux/6 -> Subsystem/1(In1), Width/1
  Data Type Conversion2/1 -> ACKSourceID/1
  Demux/1 -> Terminator2/1
  Data Type Conversion/1 -> ACKFramePara/1
  Mod/1 -> Compare To Zero/1
  Byte Unpack1/1 -> Data Type Conversion1/1
  Demux/7 -> Terminator/1
  Byte Unpack2/1 -> Data Type Conversion2/1
  Demux/5 -> Data Type Conversion4/1
  Demux/4 -> Byte Unpack2/1
  Compare To Zero/1 -> Subsystem/Enable

== system ASEToolBox2023a/ACEModule/TurnTable/8BitCheckSum1 ==
  In1 : Inport
  Add : Sum
  Bitwise AND : simulink/Logic and Bit Operations/Bitwise Operator  logicop=AND  UseBitMask=on  BitMask=hex2dec('FF')  BitMaskRealWorld=Stored Integer
      settings: LibrarySourceBlock=|
      | simulink/Quick Insert/Logic and Bit
      | Operations/Bitwise AND
  Bitwise AND1 : simulink/Logic and Bit Operations/Bitwise Operator  logicop=AND  UseBitMask=on  BitMask=hex2dec('FF')  BitMaskRealWorld=Stored Integer
      settings: LibrarySourceBlock=|
      | simulink/Quick Insert/Logic and Bit
      | Operations/Bitwise AND
  Bitwise NOT : simulink/Logic and Bit Operations/Bitwise Operator  logicop=NOT  UseBitMask=off  BitMask=bin2dec('11011001')  BitMaskRealWorld=Stored Integer
      settings: LibrarySourceBlock=|
      | simulink/Quick Insert/Logic and Bit
      | Operations/Bitwise NOT
  Constant5 : Constant
  Data Type Conversion10 : DataTypeConversion  OutDataTypeStr=uint8  SaturateOnIntegerOverflow=off  RndMeth=Floor
  Data Type Conversion11 : DataTypeConversion  OutDataTypeStr=uint16  SaturateOnIntegerOverflow=off  RndMeth=Floor
  Data Type Conversion12 : DataTypeConversion  OutDataTypeStr=uint8  SaturateOnIntegerOverflow=off  RndMeth=Floor
  Data Type Conversion8 : DataTypeConversion  OutDataTypeStr=uint32  SaturateOnIntegerOverflow=off  RndMeth=Floor
  Data Type Conversion9 : DataTypeConversion  OutDataTypeStr=uint16  SaturateOnIntegerOverflow=off  RndMeth=Floor
  Sum of Elements : Sum  Inputs=+
  Out1 : Outport
  wires:
  Bitwise NOT/1 -> Data Type Conversion9/1
  Constant5/1 -> Data Type Conversion11/1
  Sum of Elements/1 -> Bitwise AND/1
  Bitwise AND/1 -> Data Type Conversion10/1
  Add/1 -> Bitwise AND1/1
  Data Type Conversion9/1 -> Add/1
  Data Type Conversion11/1 -> Add/2
  Data Type Conversion8/1 -> Sum of Elements/1
  Data Type Conversion10/1 -> Bitwise NOT/1
  In1/1 -> Data Type Conversion8/1
  Data Type Conversion12/1 -> Out1/1
  Bitwise AND1/1 -> Data Type Conversion12/1

== system ASEToolBox2023a/Aerocraft Model/ACE Aerodynamic for 3DOF/CL ==
  alpha : Inport
  Ma : Inport  Port=2
  deltz_pp : Inport  Port=3
  Add : Sum
  CL0 : Lookup2D  RowIndex=[-2,-1,0.5,1:10]  ColumnIndex=[0.3:0.1:0.8]  Table=|  SaturateOnIntegerOverflow=off  InputSameDT=off
      | [-0.8551	-0.8635	-0.8752	-0.8919	-0.914	-0.9479
      | -0.4232	-0.4273	-0.4332	-0.4415	-0.4525	-0.4695
      | 0.2105	0.2126	0.2155	0.2196	0.2251	0.2336
      | 0.4232	0.4273	0.4332	0.4415	0.4525	0.4695
      | 0.8551	0.8635	0.8752	0.8919	0.914	0.9479
      | 1.2956	1.3082	1.3258	1.351	1.3842	1.4353
      | 1.7443	1.7612	1.7848	1.8186	1.863	1.9315
      | 2.201	2.2223	2.2519	2.2944	2.3504	2.4364
      | 2.6653	2.691	2.7269	2.7783	2.846	2.95
      | 3.1369	3.1673	3.2096	3.2701	3.3498	3.4721
      | 3.6156	3.6507	3.6996	3.7695	3.8615	4.0026
      | 4.101	4.1411	4.1967	4.2764	4.381	4.5414
      | 4.593	4.6381	4.7008	4.7905	4.9082	5.0886
      | ]
  CLDeltZ : Lookup2D  RowIndex=|  ColumnIndex=|  Table=|  SaturateOnIntegerOverflow=off  InputSameDT=off
      RowIndex=|
      | [-2
      | -1
      | 0.5
      | 1
      | 2
      | 3
      | 4
      | 5
      | 6
      | 7
      | 8
      | 9
      | 10
      | ]
      Table=|
      | [0.0513	0.0522	0.0532	0.0541	0.0541	0.0541
      | 0.0513	0.0523	0.0532	0.0542	0.0542	0.0542
      | 0.0514	0.0523	0.0533	0.0542	0.0542	0.0542
      | 0.0513	0.0523	0.0532	0.0542	0.0542	0.0542
      | 0.0513	0.0522	0.0532	0.0541	0.0541	0.0541
      | 0.0512	0.0521	0.0531	0.054	0.054	0.054
      | 0.0511	0.052	0.053	0.0539	0.0539	0.0539
      | 0.0509	0.0518	0.0528	0.0537	0.0537	0.0537
      | 0.0507	0.0516	0.0526	0.0535	0.0535	0.0535
      | 0.0505	0.0514	0.0523	0.0533	0.0533	0.0533
      | 0.0502	0.0511	0.0521	0.053	0.053	0.053
      | 0.0499	0.0508	0.0517	0.0527	0.0527	0.0527
      | 0.0496	0.0505	0.0514	0.0523	0.0523	0.0523
      | ]
      ColumnIndex=|
      | [0.3	0.4	0.5	0.6	0.7	0.8
      | ]
  Divide1 : Product  Inputs=**
  CL : Outport
  wires:
  Add/1 -> CL/1
  Divide1/1 -> Add/2
  CL0/1 -> Add/1
  CLDeltZ/1 -> Divide1/2
  alpha/1 -> CL0/1, CLDeltZ/1
  Ma/1 -> CL0/2, CLDeltZ/2
  deltz_pp/1 -> Divide1/1
